simulink model "cubesat_pd_baseline"  (R2025b)
settings: Solver=VariableStepAuto  StartTime=0.0  StopTime=30  RelTol=1e-3
values from neighbouring files (symbols this model uses):
  J = 0.05    [B1.m]
  Kd = 0.10    (= 0.1)    [B1.m]
  Ki = 0.009    [B1.m]
  Kp = 0.05    [B1.m]
  Tdist = 0.0015    [B1.m]
  theta_ref = deg2rad(45)    [B1.m]
libraries: simulink x1
settings Model: Creator=mahmo  LastModifiedBy=mahmo

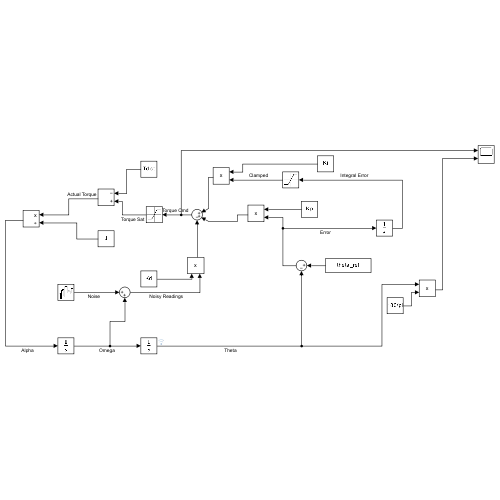
[thumbnail: Simulink's stored preview of the top-level diagram]
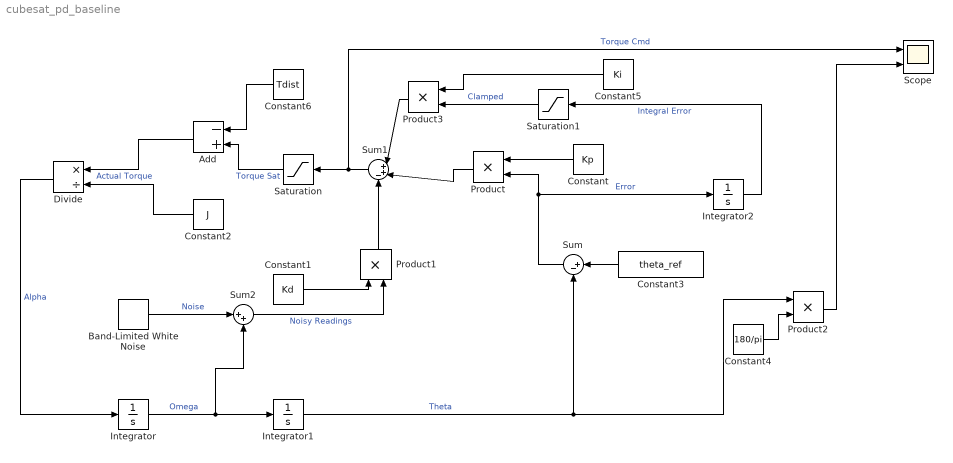
== system cubesat_pd_baseline ==
  Add : Sum  Inputs=-+
  Band-Limited White Noise : simulink/Sources/Band-Limited White Noise  Cov=(deg2rad(0.2))^2 * 0.01  Ts=0.01  seed=[23341]
  Constant : Constant  Value=Kp
  Constant1 : Constant  Value=Kd
  Constant2 : Constant  Value=J
  Constant3 : Constant  Value=theta_ref
  Constant4 : Constant  Value=180/pi
  Constant5 : Constant  Value=Ki
  Constant6 : Constant  Value=Tdist
  Divide : Product  Inputs=*/
  Integrator : Integrator
  Integrator1 : Integrator
  Integrator2 : Integrator
  Product{,1..3} (4 alike) : Product
  Saturation : Saturate  UpperLimit=0.005  LowerLimit=-0.005
  Saturation1 : Saturate  UpperLimit=0.22  LowerLimit=-0.22
  Scope : Scope  NumInputPorts=2
      settings: ActiveDisplayYMinimum=30.013221932114014  ActiveDisplayYMaximum=46.824824572698546
  Sum : Sum  Inputs=|+-
  Sum1 : Sum  Inputs=|++-
  Sum2 : Sum  Inputs=|++
  wires:
  Integrator/1 -> Integrator1/1, Sum2/2  "Omega"
  Integrator1/1 -> Product2/1, Sum/2  "Theta"
  Divide/1 -> Integrator/1  "Alpha"
  Sum/1 -> Integrator2/1, Product/2  "Error"
  Constant3/1 -> Sum/1
  Constant/1 -> Product/1
  Product/1 -> Sum1/2
  Product1/1 -> Sum1/3
  Constant1/1 -> Product1/1
  Sum1/1 -> Scope/1, Saturation/1  "Torque Cmd"
  Constant2/1 -> Divide/2
  Constant4/1 -> Product2/2
  Product2/1 -> Scope/2
  Integrator2/1 -> Saturation1/1  "Integral Error"
  Constant5/1 -> Product3/1
  Product3/1 -> Sum1/1
  Constant6/1 -> Add/1
  Saturation/1 -> Add/2  "Torque Sat"
  Add/1 -> Divide/1  "Actual Torque"
  Band-Limited White Noise/1 -> Sum2/1  "Noise"
  Sum2/1 -> Product1/2  "Noisy Readings"
  Saturation1/1 -> Product3/2  "Clamped"
